simulink model "fft_wideband_real_test"  (Simulink 7.4)
settings: Solver=VariableStepDiscrete  StartTime=0.0  StopTime=150  RelTol=1e-3
libraries: xbsIndex_r4 x739, casper_library_misc x48, casper_library_delays x8, casper_library_ffts_twiddle x1, simulink x1
(part 1 of 7)
settings Model: Creator=User  LastModifiedBy=wjm
settings OptimizationCC: InitFltsAndDblsToZero=on

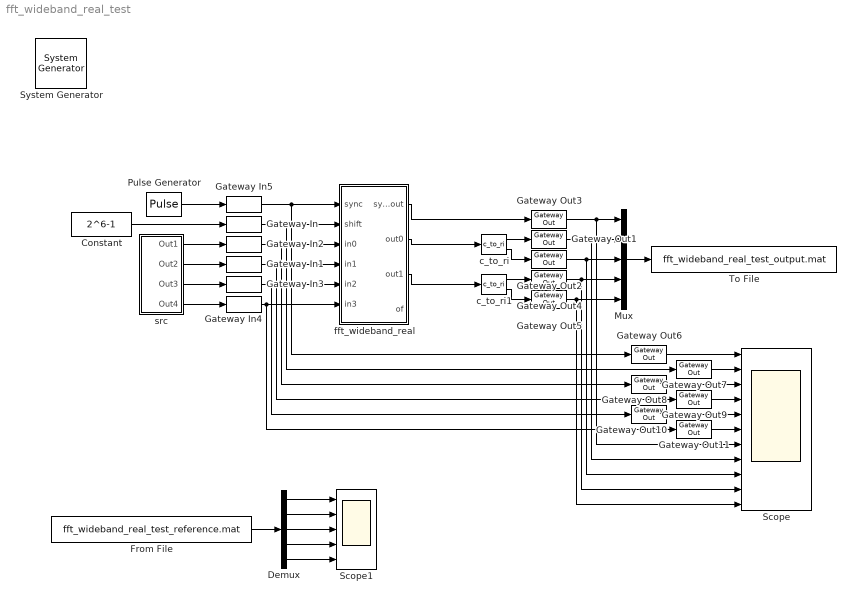
== system fft_wideband_real_test ==
  " System Generator" : xbsIndex_r4/ System Generator  Tag=genX  SystemSampleTime=-1  xilinxfamily=virtex5  part=xc5vsx95t  speed=-1  package=ff1136  synthesis_tool=XST  clock_wrapper=Clock Enables  directory=./netlist  testbench=off  simulink_period=1  sysclk_period=100  dcm_input_clock_period=100  incr_netlist=off  trim_vbits=Everywhere in SubSystem  dbl_ovrd=According to Block Masks  core_generation=According to Block Masks  run_coregen=off  deprecated_control=off  eval_field=0  block_type=sysgen
      settings: block_version=10.1.1
  Constant : Constant  Value=2^6-1  OutDataType=sfix(16)  OutScaling=2^0
  Demux : Demux  Outputs=5
  From File : FromFile  FileName=fft_wideband_real_test_reference.mat  SampleTime=1
  Gateway In : xbsIndex_r4/Gateway In  arith_type=Unsigned  n_bits=6  bin_pt=0  quantization=Truncate  overflow=Wrap  period=1  dbl_ovrd=off  timing_constraint=None  locs_specified=off  LOCs={}  hdl_port=on  block_type=gatewayin
      settings: infoedit="Gateway in block.  Converts inputs of type Simulink integer, double and fixed point to  Xilinx fixed point type.<P><P>Hardware notes:  In hardware these blocks become top level input ports."  block_version=10.1.1
  Gateway In{1..4} (4 alike) : xbsIndex_r4/Gateway In  arith_type="Signed  (2's comp)"  n_bits=12  bin_pt=11  quantization=Truncate  overflow=Wrap  period=1  dbl_ovrd=off  timing_constraint=None  locs_specified=off  LOCs={}  hdl_port=on  block_type=gatewayin
      settings: infoedit="Gateway in block.  Converts inputs of type Simulink integer, double and fixed point to  Xilinx fixed point type.<P><P>Hardware notes:  In hardware these blocks become top level input ports."  block_version=10.1.1
  Gateway In5 : xbsIndex_r4/Gateway In  arith_type=Boolean  n_bits=16  bin_pt=14  quantization="Round  (unbiased: +/- Inf)"  overflow=Saturate  period=1  dbl_ovrd=off  timing_constraint=None  locs_specified=off  LOCs={}  hdl_port=on  block_type=gatewayin
      settings: infoedit="Gateway in block.  Converts inputs of type Simulink integer, double and fixed point to  Xilinx fixed point type.<P><P>Hardware notes:  In hardware these blocks become top level input ports."  block_version=10.1.1
  Gateway Out{1..11} (11 alike) : xbsIndex_r4/Gateway Out  hdl_port=on  timing_constraint=None  locs_specified=off  LOCs={}  block_type=gatewayout
      settings: infoedit="Gateway out block.  Converts Xilinx fixed point inputs into ouputs of type Simulink integer, double, or fixed point.<P><P>Hardware notes:  In hardware these blocks become top level output ports or are discarded, depending on how they are configured."  block_version=10.1.1
  Mux : Mux  Inputs=5
  Pulse Generator : DiscretePulseGenerator  Amplitude=1  Period=2^6  PulseWidth=1  PhaseDelay=13  SampleTime=1
  Scope : Scope  NumInputPorts=11
      settings: TimeRange=256  YMin=-5~-5~-5~-5~-5~-5~-5~-5~-5~-5~-5  YMax=5~5~5~5~5~5~5~5~5~5~5
  Scope1 : Scope  NumInputPorts=5
      settings: YMin=-5~-5~-5~-5~-5  YMax=5~5~5~5~5
  To File : ToFile  Filename=fft_wideband_real_test_output.mat  MatrixName=output
  c_to_ri : casper_library_misc/c_to_ri  SystemSampleTime=-1  n_bits=12  bin_pt=11
      settings: AttributesFormatString=12_11 r/i
  c_to_ri1 : casper_library_misc/c_to_ri  SystemSampleTime=-1  n_bits=12  bin_pt=11
      settings: AttributesFormatString=12_11 r/i
  fft_wideband_real : Subsystem  AncestorBlock=casper_library_ffts/fft_wideband_real  mask(fft_wideband_real){FFTSize=5, input_bit_width=12, coeff_bit_width=12, n_inputs=2, quantization=Round  (unbiased: Even Values), overflow=Saturate, add_latency=2, mult_latency=2, bram_latency=1, conv_latency=2, arch=Virtex5, opt_target=multipliers, coeffs_bit_limit=8, delays_bit_limit=8, specify_mult=on, mult_spec=getfield( getfield( get_param( gcb,'UserData' ), 'parameters'),'mult_spec'), dsp48_adders=on}
      mask prompts: FFTSize "Size of FFT: (2^?)"; input_bit_width "Input/Output Bit Width"; coeff_bit_width "Coefficient Bit Width"; n_inputs "Number of Simultaneous Inputs: (2^?)"; quantization "Quantization Behavior"; overflow "Overflow Behavior"; add_latency "Add Latency"; mult_latency "Mult Latency"; bram_latency "BRAM Latency"; conv_latency "Convert latency"; arch "Architecture"; opt_target "Use less"; coeffs_bit_limit "Number bits above which to store stage's coefficients in BRAM (2^? bits)"; delays_bit_limit "Number bits above which to store stage's delays in BRAM (2^? bits)"; specify_mult "Specify multiplier use (behavioral HDL if not specified)"; mult_spec "Multiplier specification (0=core, 1=embedded, 2=behavioural) (left=1st stage)"; dsp48_adders "DSP48 adders in butterfly"
      mask init:
      | fft_wideband_real_init(gcb,...
      |     'FFTSize', FFTSize,...
      |     'input_bit_width', input_bit_width,...
      |     'coeff_bit_width', coeff_bit_width,...
      |     'n_inputs', n_inputs,...
      |     'quantization', quantization,...
      |     'overflow', overflow,...
      |     'add_latency', add_latency,...
      |     'mult_latency', mult_latency,...
      |     'bram_latency', bram_latency,...
      |     'conv_latency', conv_latency, ...
      |     'arch', arch, ...
      |     'opt_target', opt_target, ...
      |     'coeffs_bit_limit', coeffs_bit_limit, ...
      |     'delays_bit_limit', delays_bit_limit, ...    
      |     'specify_mult', specify_mult,...
      |     'mult_spec', mult_spec, ...
      |     'dsp48_adders', dsp48_adders);
      settings: AttributesFormatString=|
      | 5 stages
      | (12,12)
      | Round  (unbiased: Even Values)
      | Saturate
      mask Help: eval('xlWeb(''http://casper.berkeley.edu/wiki/Fft_wideband_real'')')
      mask StyleString: edit,edit,edit,edit,popup(Truncate|Round  (unbiased: +/- Inf)|Round  (unbiased: Even Values)),popup(Wrap|Saturate|Error),edit,edit,edit,edit,popup(Virtex2Pro|Virtex5),popup(logic|multipliers),edit,edit,checkbox,edit,checkbox
      mask CallbackString:
      | % fft_size = eval(get_param(gcb, 'FFTSize'));
      | % old_vec = eval(get_param(gcb, 'mult_spec'));
      | 
      | % vec = 2.*ones(1,fft_size);
      | % old_size = length(old_vec);
      | 
      | % if(old_size <= fft_size),
      | %    size = old_size;
      | % else,
      | %     size = fft_size;
      | % end
      | 
      | % for n = 1:size, vec(n) = old_vec(n); end
      | % set_param(gcb, 'mult_spec', mat2str(vec));||||||||||fft_callback_arch(gcb);||||specify_mult = get_param(gcb,'specify_mult');
      | visibs = get_param(gcb, 'MaskVisibilities');
      | enables = get_param(gcb, 'MaskEnables');
      | enables{16} = 'on';
      | if( strcmp(specify_mult,'off')), visibs{16} = 'off';
      | else, visibs{16} = 'on';
      | end
      | set_param(gcb, 'MaskEnables', enables);
      | set_param(gcb, 'MaskVisibilities', visibs);
      | |% vec = eval( get_param(gcb, 'mult_spec'));
      | % vec_size = length(vec);
      | % fft_size = eval( get_param(gcb, 'FFTSize'));
      | % new_vec = 2.*ones(1, fft_size);
      | 
      | % if(vec_size <= fft_size), size = vec_size;
      | % else size = fft_size;
      | % end
      | 
      | % for n=1:size
      | %     new_vec(n) = vec(n);
      | % end
      | % set_param(gcb, 'mult_spec', mat2str(new_vec));|fft_callback_dsp48_adders(gcb);
  src : Subsystem
  wires:
  Pulse Generator/1 -> Gateway In5/1
  Constant/1 -> Gateway In/1
  src/1(Out1) -> Gateway In2/1
  src/2(Out2) -> Gateway In1/1
  src/3(Out3) -> Gateway In3/1
  src/4(Out4) -> Gateway In4/1
  Gateway In2/1 -> Gateway Out8/1, fft_wideband_real/3(in0)
  Gateway In1/1 -> Gateway Out9/1, fft_wideband_real/4(in1)
  Gateway In3/1 -> Gateway Out10/1, fft_wideband_real/5(in2)
  Gateway In4/1 -> Gateway Out11/1, fft_wideband_real/6(in3)
  Gateway In/1 -> Gateway Out7/1, fft_wideband_real/2(shift)
  Gateway In5/1 -> Gateway Out6/1, fft_wideband_real/1(sync)
  fft_wideband_real/1(sync_out) -> Gateway Out3/1
  fft_wideband_real/2(out0) -> c_to_ri/1
  fft_wideband_real/3(out1) -> c_to_ri1/1
  c_to_ri/1 -> Gateway Out1/1
  c_to_ri/2 -> Gateway Out2/1
  c_to_ri1/1 -> Gateway Out4/1
  c_to_ri1/2 -> Gateway Out5/1
  Gateway Out3/1 -> Mux/1, Scope/7
  Gateway Out1/1 -> Mux/2, Scope/8
  Gateway Out2/1 -> Mux/3, Scope/9
  Gateway Out4/1 -> Mux/4, Scope/10
  Gateway Out5/1 -> Mux/5, Scope/11
  Mux/1 -> To File/1
  Gateway Out6/1 -> Scope/1
  Gateway Out7/1 -> Scope/2
  Gateway Out8/1 -> Scope/3
  Gateway Out9/1 -> Scope/4
  Gateway Out10/1 -> Scope/5
  Gateway Out11/1 -> Scope/6
  From File/1 -> Demux/1
  Demux/1 -> Scope1/1
  Demux/2 -> Scope1/2
  Demux/3 -> Scope1/3
  Demux/4 -> Scope1/4
  Demux/5 -> Scope1/5

== system fft_wideband_real_test/fft_wideband_real ==
  sync : Inport
  shift : Inport  Port=2
  in0 : Inport  Port=3
  in1 : Inport  Port=4
  in2 : Inport  Port=5
  in3 : Inport  Port=6
  fft_biplex_real_4x0 : Subsystem  AncestorBlock=casper_library_ffts/fft_biplex_real_4x  mask(fft_biplex_real_4x){FFTSize=3, input_bit_width=12, coeff_bit_width=12, quantization=Round  (unbiased: Even Values), overflow=Saturate, add_latency=2, mult_latency=2, bram_latency=1, conv_latency=2, arch=Virtex5, opt_target=multipliers, coeffs_bit_limit=8, delays_bit_limit=8, specify_mult=on, mult_spec=[0                                      1                                      2], dsp48_adders=on}
      mask prompts: FFTSize "Size of FFT: (2^? pnts)"; input_bit_width "Input/Output Bit Width"; coeff_bit_width "Coefficient Bit Width"; quantization "Quantization Behavior"; overflow "Overflow Behavior"; add_latency "Add Latency"; mult_latency "Mult Latency"; bram_latency "BRAM Latency"; conv_latency "Convert latency"; arch "Architecture"; opt_target "Use less"; coeffs_bit_limit "Number bits above which to store stage's coefficients in BRAM (2^? bits)"; delays_bit_limit "Number bits above which to implement stage's delays in BRAM (2^? bits)"; specify_mult "Specify multiplier use (behavioral HDL if not specified)"; mult_spec "Multiplier specification (0=core, 1=embedded, 2=behavioural) (left=1st stage)"; dsp48_adders "DSP48 adders in butterfly"
      mask init:
      | fft_biplex_real_4x_init(gcb, ...
      |     'FFTSize', FFTSize, ...
      |     'input_bit_width', input_bit_width, ...
      |     'coeff_bit_width', coeff_bit_width, ...
      |     'quantization', quantization, ...
      |     'overflow', overflow, ...
      |     'add_latency', add_latency, ...
      |     'mult_latency', mult_latency, ...
      |     'bram_latency', bram_latency, ...
      |     'conv_latency', conv_latency, ...
      |     'arch', arch, ...
      |     'opt_target', opt_target, ...
      |     'coeffs_bit_limit', coeffs_bit_limit, ...
      |     'delays_bit_limit', delays_bit_limit, ...    
      |     'specify_mult', specify_mult, ...
      |     'mult_spec', mult_spec, ...
      |     'dsp48_adders', dsp48_adders);
      settings: AttributesFormatString=|
      | Virtex5
      | 3 stages
      | [12,12]
      | Round  (unbiased: Even Values)
      | Saturate
      mask Help: eval('xlWeb(''http://casper.berkeley.edu/wiki/Fft_biplex_real_4x'')')
      mask StyleString: edit,edit,edit,popup(Truncate|Round  (unbiased: +/- Inf)|Round  (unbiased: Even Values)),popup(Wrap|Saturate|Error),edit,edit,edit,edit,popup(Virtex2Pro|Virtex5),popup(logic|multipliers),edit,edit,checkbox,edit,checkbox
      mask CallbackString:
      | % fft_size = eval(get_param(gcb, 'FFTSize'));
      | % old_vec = eval(get_param(gcb, 'mult_spec'));
      | 
      | % vec = 2.*ones(1,fft_size);
      | % old_size = length(old_vec);
      | 
      | % if(old_size <= fft_size),
      | %     size = old_size;
      | % else,
      | %     size = fft_size;
      | % end
      | 
      | % for n = 1:size, vec(n) = old_vec(n); end
      | % set_param(gcb, 'mult_spec', mat2str(vec));|||||||||fft_callback_arch(gcb);||||specify_mult = get_param(gcb,'specify_mult');
      | visibs = get_param(gcb, 'MaskVisibilities');
      | enables = get_param(gcb, 'MaskEnables');
      | enables{15} = 'on';
      | if( strcmp(specify_mult,'off')), visibs{15} = 'off';
      | else, visibs{15} = 'on';
      | end
      | set_param(gcb, 'MaskVisibilities', visibs);
      | set_param(gcb, 'MaskEnables', enables);
      | |% vec = eval( get_param(gcb, 'mult_spec'));
      | % vec_size = length(vec);
      | % fft_size = eval( get_param(gcb, 'FFTSize'));
      | % new_vec = 2.*ones(1, fft_size);
      | 
      | % if(vec_size <= fft_size), size = vec_size;
      | % else size = fft_size;
      | % end
      | 
      | % for n=1:size
      | %    new_vec(n) = vec(n);
      | % end
      | % set_param(gcb, 'mult_spec', mat2str(new_vec));|fft_callback_dsp48_adders(gcb);
  fft_direct : Subsystem  AncestorBlock=casper_library_ffts/fft_direct  mask(fft_direct){FFTSize=2, input_bit_width=12, coeff_bit_width=12, add_latency=2, mult_latency=2, bram_latency=1, conv_latency=2, quantization=Round  (unbiased: Even Values), overflow=Saturate, map_tail=on, LargerFFTSize=5, StartStage=4, arch=Virtex5, opt_target=multipliers, coeffs_bit_limit=8, specify_mult=on, mult_spec=[0                                      1], dsp48_adders=on}
      mask prompts: FFTSize "Size of FFT: (2^?)"; input_bit_width "Input/Output Bit Width"; coeff_bit_width "Coefficient Bit Width"; add_latency "Add Latency"; mult_latency "Mult Latency"; bram_latency "BRAM Latency"; conv_latency "Convert latency"; quantization "Quantization Behavior"; overflow "Overflow Behavior"; map_tail "Map Tail of Larger FFT"; LargerFFTSize "Size of Larger FFT (2^?):"; StartStage "Start Stage of Map Tail:"; arch "Architecture"; opt_target "Use less"; coeffs_bit_limit "Number bits above which to store stage's coefficients in BRAM (2^? bits)"; specify_mult "Specify multiplier use (behavioural HDL if not specified)"; mult_spec "Multiplier specification (0=core, 1=behavioural HDL, 2=embedded) (left=1st stage)"; dsp48_adders "DSP48 adders in butterfly"
      mask help:
      | Implements an N-point FFT with the classic
      | butterfly structure with N inputs and N outputs
      mask init:
      | fft_direct_init(gcb,...
      |     'FFTSize', FFTSize, ...
      |     'input_bit_width', input_bit_width, ...
      |     'coeff_bit_width', coeff_bit_width, ...
      |     'add_latency', add_latency, ...
      |     'mult_latency', mult_latency, ...
      |     'bram_latency', bram_latency, ...
      |     'conv_latency', conv_latency, ...
      |     'quantization', quantization, ...
      |     'overflow', overflow, ...
      |     'map_tail', map_tail, ...
      |     'LargerFFTSize', LargerFFTSize, ...
      |     'StartStage', StartStage, ...
      |     'arch', arch, ...
      |     'opt_target', opt_target, ...
      |     'coeffs_bit_limit', coeffs_bit_limit, ...
      |     'specify_mult', specify_mult, ...
      |     'mult_spec', mult_spec, ...
      |     'dsp48_adders', dsp48_adders);
      settings: AttributesFormatString=|
      | Virtex5
      | stages [4  5] of 5
      | [12,12]
      | Round  (unbiased: Even Values)
      | Saturate
      mask StyleString: edit,edit,edit,edit,edit,edit,edit,popup(Truncate|Round  (unbiased: +/- Inf)|Round  (unbiased: Even Values)),popup(Wrap|Saturate|Error),checkbox,edit,edit,popup(Virtex2Pro|Virtex5),popup(logic|multipliers),edit,checkbox,edit,checkbox
      mask CallbackString:
      | % fft_size = eval(get_param(gcb, 'FFTSize'));
      | % old_vec = eval(get_param(gcb, 'mult_spec'));
      | 
      | % vec = 2.*ones(1,fft_size);
      | % old_size = length(old_vec);
      | 
      | % if(old_size <= fft_size),
      | %     size = old_size;
      | % else,
      | %     size = fft_size;
      | % end
      | 
      | % for n = 1:size, vec(n) = old_vec(n); end
      | % set_param(gcb, 'mult_spec', mat2str(vec));|||||||||map_tail = get_param(gcb,'map_tail');
      | visibs = get_param(gcb, 'MaskVisibilities');
      | if( strcmp(map_tail,'off')),
      |     visibs{11} = 'off';
      |     visibs{12} = 'off';
      | else,
      |     visibs{11} = 'on';
      |     visibs{12} = 'on';
      | end
      | set_param(gcb, 'MaskVisibilities', visibs);
      | |||fft_callback_arch(gcb);|||specify_mult = get_param(gcb,'specify_mult');
      | visibs = get_param(gcb, 'MaskVisibilities');
      | if( strcmp(specify_mult,'off')), visibs{17} = 'off';
      | else, visibs{17} = 'on';
      | end
      | set_param(gcb, 'MaskVisibilities', visibs);
      | |% vec = eval( get_param(gcb, 'mult_spec'));
      | % vec_size = length(vec);
      | % fft_size = eval( get_param(gcb, 'FFTSize'));
      | % new_vec = 2.*ones(1, fft_size);
      | 
      | % if(vec_size <= fft_size), size = vec_size;
      | % else size = fft_size;
      | % end
      | 
      | % for n=1:size
      | %     new_vec(n) = vec(n);
      | % end
      | % set_param(gcb, 'mult_spec', mat2str(new_vec));|fft_callback_dsp48_adders(gcb);
  fft_unscrambler : Subsystem  AncestorBlock=casper_library_ffts/fft_unscrambler  mask(fft_unscrambler){FFTSize=4, n_inputs=1, bram_latency=1}
      mask prompts: FFTSize "Size of FFT: (2^?)"; n_inputs "Number of Simultaneous Inputs: (2^?)"; bram_latency "BRAM Latency"
      mask init:
      | fft_unscrambler_init(gcb,...
      |     'FFTSize',FFTSize,... 
      |     'n_inputs', n_inputs,...
      |     'bram_latency', bram_latency);
      settings: AttributesFormatString=FFTSize=4, n_inputs=1
  of_or : xbsIndex_r4/Logical  logical_function=OR  inputs=2  en=off  latency=1  precision=Full  arith_type=Unsigned  n_bits=16  bin_pt=0  align_bp=on  dbl_ovrd=off  block_type=logical
      settings: block_version=11.4
  slice : xbsIndex_r4/Slice  nbits=2  boolean_output=off  mode=Lower Bit Location + Width  bit1=0  base1=MSB of Input  bit0=3  base0=LSB of Input  dbl_ovrd=off  block_type=slice
  sync_out : Outport
  out0 : Outport  Port=2
  out1 : Outport  Port=3
  of : Outport  Port=4
  wires:
  in0/1 -> fft_biplex_real_4x0/1(pol1)
  in1/1 -> fft_biplex_real_4x0/2(pol2)
  in2/1 -> fft_biplex_real_4x0/3(pol3)
  in3/1 -> fft_biplex_real_4x0/4(pol4)
  shift/1 -> fft_biplex_real_4x0/6(shift), slice/1
  sync/1 -> fft_biplex_real_4x0/5(sync)
  fft_biplex_real_4x0/5(of) -> of_or/2
  slice/1 -> fft_direct/2(shift)
  fft_biplex_real_4x0/6(sync_out) -> fft_direct/1(sync)
  fft_biplex_real_4x0/1(pol1_out) -> fft_direct/3(in0)
  fft_biplex_real_4x0/2(pol2_out) -> fft_direct/4(in1)
  fft_biplex_real_4x0/3(pol3_out) -> fft_direct/5(in2)
  fft_biplex_real_4x0/4(pol4_out) -> fft_direct/6(in3)
  fft_direct/6(of) -> of_or/1
  of_or/1 -> of/1
  fft_direct/1(sync_out) -> fft_unscrambler/1(sync)
  fft_unscrambler/1(sync_out) -> sync_out/1
  fft_direct/2(out0) -> fft_unscrambler/2(In1)
  fft_unscrambler/2(Out1) -> out0/1
  fft_direct/3(out1) -> fft_unscrambler/3(In2)
  fft_unscrambler/3(Out2) -> out1/1

== system fft_wideband_real_test/src ==
  Band-Limited White Noise : simulink/Sources/Band-Limited White Noise  SystemSampleTime=-1  Cov=[0.001]  Ts=1  seed=[23341]
  Constant : Constant  Value=0  OutDataType=sfix(16)  OutScaling=2^0
  Pulse Generator1 : DiscretePulseGenerator  Amplitude=0.75  Period=2^5  PulseWidth=1  PhaseDelay=14  SampleTime=1
  Pulse Generator2 : DiscretePulseGenerator  Amplitude=0.5  Period=2^6  PulseWidth=1  PhaseDelay=15  SampleTime=1
  Sine Wave : Sin  SineType=Sample based  Amplitude=0.125  Bias=0  Frequency=1  Phase=0  Samples=8  SampleTime=1  Offset=0
  Out1 : Outport
  Out2 : Outport  Port=2
  Out3 : Outport  Port=3
  Out4 : Outport  Port=4
  wires:
  Pulse Generator2/1 -> Out4/1, Out3/1
  Pulse Generator1/1 -> Out1/1, Out2/1

== system fft_wideband_real_test/fft_wideband_real/fft_biplex_real_4x0 ==
  pol1 : Inport  OutDataType=sfix(16)  OutScaling=2^0
  pol2 : Inport  Port=2  OutDataType=sfix(16)  OutScaling=2^0
  pol3 : Inport  Port=3  OutDataType=sfix(16)  OutScaling=2^0
  pol4 : Inport  Port=4  OutDataType=sfix(16)  OutScaling=2^0
  sync : Inport  Port=5  OutDataType=sfix(16)  OutScaling=2^0
  shift : Inport  Port=6  OutDataType=sfix(16)  OutScaling=2^0
  bi_real_unscr_4x : Subsystem  mask{FFTSize=3, bram_latency=1}
      mask prompts: FFTSize "Size of FFT (2^?):"; bram_latency "BRAM Latency"
      mask init:
      | blk = gcb;
      | if same_state(blk, 'FFTSize', FFTSize, 'bram_latency', bram_latency), return, end
      | set_param([blk,'/reorder'],'map', mat2str(bit_reverse(0:2^(FFTSize-1)-1, FFTSize-1)));
      | set_param([blk,'/reorder'],'bram_latency', num2str(bram_latency));
      | set_param([blk,'/reorder1'],'map', mat2str(bit_reverse(2^(FFTSize-1)-1:-1:0, FFTSize-1)));
      | set_param([blk,'/reorder1'],'bram_latency', num2str(bram_latency));
      | set_param([blk,'/reorder2'],'map', mat2str(2^(FFTSize-1)-1:-1:0));
      | set_param([blk,'/reorder2'],'bram_latency', num2str(bram_latency));
      | save_state(blk, 'FFTSize', FFTSize, 'bram_latency', bram_latency);
  biplex_core : Subsystem  AncestorBlock=casper_library_ffts/biplex_core  mask(biplex_core){FFTSize=3, input_bit_width=12, coeff_bit_width=12, quantization=Round  (unbiased: Even Values), overflow=Saturate, add_latency=2, mult_latency=2, bram_latency=1, conv_latency=2, arch=Virtex5, opt_target=multipliers, coeffs_bit_limit=8, delays_bit_limit=8, specify_mult=on, mult_spec=[0                                      1                                      2], dsp48_adders=on}
      mask prompts: FFTSize "Size of FFT: (2^? pnts)"; input_bit_width "Input/Output Bit Width"; coeff_bit_width "Coefficient Bit Width"; quantization "Quantization Behavior"; overflow "Overflow Behavior"; add_latency "Add Latency"; mult_latency "Mult Latency"; bram_latency "BRAM Latency"; conv_latency "Convert latency"; arch "Architecture"; opt_target "Use less"; coeffs_bit_limit "Number bits above which to store stage's coefficients in BRAM (2^? bits)"; delays_bit_limit "Number bits above which to implent stage's delays in BRAM (2^? bits)"; specify_mult "Specify multiplier use (behavioural HDL if not specified)"; mult_spec "Multiplier specification (0=core, 1=embedded, 2=behavioural) (left=1st stage)"; dsp48_adders "Use DSP48s for adders"
      mask init:
      | biplex_core_init(gcb,...
      |     'FFTSize', FFTSize,...
      |     'input_bit_width', input_bit_width,...
      |     'coeff_bit_width', coeff_bit_width,...
      |     'quantization', quantization,...
      |     'overflow', overflow,...
      |     'add_latency', add_latency,...
      |     'mult_latency', mult_latency,...
      |     'bram_latency', bram_latency,...
      |     'conv_latency', conv_latency, ...
      |     'arch', arch, ...
      |     'opt_target', opt_target, ...
      |     'coeffs_bit_limit', coeffs_bit_limit, ...
      |     'delays_bit_limit', delays_bit_limit, ...
      |     'specify_mult', specify_mult, ...
      |     'mult_spec', mult_spec, ...
      |     'dsp48_adders', dsp48_adders );
      settings: AttributesFormatString=|
      | 3 stages
      | reduce multipliers
      | Virtex5
      mask StyleString: edit,edit,edit,popup(Truncate|Round  (unbiased: +/- Inf)|Round  (unbiased: Even Values)),popup(Wrap|Saturate|Error),edit,edit,edit,edit,popup(Virtex2Pro|Virtex5),popup(logic|multipliers),edit,edit,checkbox,edit,checkbox
      mask CallbackString:
      | % fft_size = eval(get_param(gcb, 'FFTSize'));
      | % old_vec = eval(get_param(gcb, 'mult_spec'));
      | 
      | % vec = 2.*ones(1,fft_size);
      | % old_size = length(old_vec);
      | 
      | % if(old_size <= fft_size),
      | %    size = old_size;
      | % else,
      | %     size = fft_size;
      | % end
      | 
      | % for n = 1:size, vec(n) = old_vec(n); end
      | % set_param(gcb, 'mult_spec', mat2str(vec));|||||||||fft_callback_arch(gcb);||||specify_mult = get_param(gcb,'specify_mult');
      | visibs = get_param(gcb,'MaskVisibilities');
      | if( strcmp(specify_mult,'off')), visibs{15} = 'off';
      | else, visibs{15} = 'on';
      | end
      | set_param(gcb, 'MaskVisibilities', visibs);
      | enables = get_param(gcb,'MaskVisibilities');
      | enables{15} = 'on';
      | set_param(gcb, 'MaskEnables', enables);
      | |% vec = eval( get_param(gcb, 'mult_spec'));
      | % vec_size = length(vec);
      | % fft_size = eval( get_param(gcb, 'FFTSize'));
      | % new_vec = 2.*ones(1, fft_size);
      | 
      | % if(vec_size <= fft_size), size = vec_size;
      | % else size = fft_size;
      | % end
      | 
      | % for n=1:size
      | %     new_vec(n) = vec(n);
      | % end
      | % set_param(gcb, 'mult_spec', mat2str(new_vec));|fft_callback_dsp48_adders(gcb);
  ri_to_c : Subsystem
  ri_to_c1 : Subsystem
  pol1_out : Outport  OutDataType=sfix(16)  OutScaling=2^0
  pol2_out : Outport  Port=2  OutDataType=sfix(16)  OutScaling=2^0
  pol3_out : Outport  Port=3  OutDataType=sfix(16)  OutScaling=2^0
  pol4_out : Outport  Port=4  OutDataType=sfix(16)  OutScaling=2^0
  of : Outport  Port=5  OutDataType=sfix(16)  OutScaling=2^0
  sync_out : Outport  Port=6  OutDataType=sfix(16)  OutScaling=2^0
  wires:
  bi_real_unscr_4x/5(sync_out) -> sync_out/1
  bi_real_unscr_4x/4(pol4_out) -> pol4_out/1
  bi_real_unscr_4x/3(pol3_out) -> pol3_out/1
  bi_real_unscr_4x/2(pol2_out) -> pol2_out/1
  bi_real_unscr_4x/1(pol1_out) -> pol1_out/1
  shift/1 -> biplex_core/4(shift)
  sync/1 -> biplex_core/3(sync)
  pol4/1 -> ri_to_c1/2(im)
  ri_to_c1/1(c) -> biplex_core/2(pol2)
  pol3/1 -> ri_to_c1/1(re)
  pol2/1 -> ri_to_c/2(im)
  ri_to_c/1(c) -> biplex_core/1(pol1)
  pol1/1 -> ri_to_c/1(re)
  biplex_core/3(of) -> of/1
  biplex_core/1(out1) -> bi_real_unscr_4x/1(even)
  biplex_core/2(out2) -> bi_real_unscr_4x/2(odd)
  biplex_core/4(sync_out) -> bi_real_unscr_4x/3(sync)

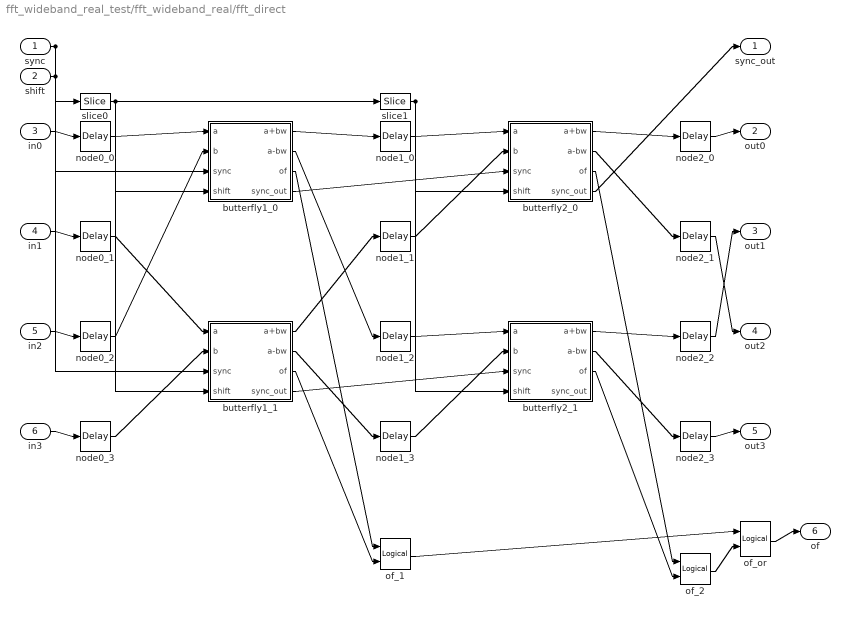
== system fft_wideband_real_test/fft_wideband_real/fft_direct ==
  sync : Inport
  shift : Inport  Port=2
  in0 : Inport  Port=3
  in1 : Inport  Port=4
  in2 : Inport  Port=5
  in3 : Inport  Port=6
  butterfly1_0 : Subsystem  AncestorBlock=casper_library_ffts/butterfly_direct  mask(butterfly_direct){biplex=off, FFTSize=5, Coeffs=getfield( getfield( get_param( gcb,'UserData' ), 'parameters'),'Coeffs'), StepPeriod=0, coeffs_bram=off, coeff_bit_width=12, input_bit_width=12, bram_latency=1, add_latency=2, mult_latency=2, conv_latency=2, quantization=Round  (unbiased: Even Values), overflow=Saturate, arch=Virtex5, opt_target=multipliers, use_hdl=off, use_embedded=off, dsp48_adders=on}
      mask prompts: biplex "Used in biplex FFT"; FFTSize "Size of FFT: (2^?)"; Coeffs "Coefficients: (0 to 2^(FFTSize-1)-1)"; StepPeriod "Coefficient Step Period: (2^?)"; coeffs_bram "Implement coefficients in BRAM"; coeff_bit_width "Coefficient Bit Width"; input_bit_width "Input/Output Bit Width:"; bram_latency "BRAM Latency"; add_latency "Add Latency"; mult_latency "Mult Latency"; conv_latency "Convert latency"; quantization "Quantization Behavior"; overflow "Overflow Behavior"; arch "Architecture"; opt_target "Use less"; use_hdl "Use behavioural HDL for multipliers"; use_embedded "Use embedded multipliers"; dsp48_adders "Use DSP48s for adders"
      mask init:
      | butterfly_direct_init(gcb,...
      |     'biplex', biplex,...
      |     'FFTSize', FFTSize,...
      |     'Coeffs', Coeffs,...
      |     'coeff_bit_width', coeff_bit_width,...
      |     'StepPeriod', StepPeriod,...
      |     'input_bit_width', input_bit_width,...
      |     'add_latency', add_latency,...
      |     'mult_latency', mult_latency,...
      |     'bram_latency', bram_latency,...
      |     'conv_latency', conv_latency, ...
      |     'coeffs_bram', coeffs_bram,...    
      |     'quantization', quantization,...
      |     'overflow', overflow,...
      |     'arch', arch,...
      |     'opt_target', opt_target,...
      |     'use_hdl', use_hdl,...
      |     'use_embedded', use_embedded,...
      |     'dsp48_adders', dsp48_adders);
      settings: AttributesFormatString=|
      | twiddle_general_3mult
      | coeffs in slices
      mask StyleString: checkbox,edit,edit,edit,checkbox,edit,edit,edit,edit,edit,edit,popup(Truncate|Round  (unbiased: +/- Inf)|Round  (unbiased: Even Values)),popup(Wrap|Saturate|Error),popup(Virtex2Pro|Virtex5),popup(logic|multipliers),checkbox,checkbox,checkbox
      mask CallbackString:
      | ||%coeffs = eval(get_param(gcb,'Coeffs'));
      | %visibs = get_param(gcb,'MaskVisibilities');
      | %if length(coeffs) == 1,
      | %    visibs{4} = 'off'; visibs{5} = 'off';
      | %    visibs{6} = 'off';
      | %else
      | %    visibs{4} = 'on';
      | %    visibs{5} = 'on'; visibs{6} = 'on';
      | %end
      | %set_param(gcb, 'MaskVisibilities', visibs);|%coeffs = eval(get_param(gcb,'Coeffs'));
      | %visibs = get_param(gcb,'MaskVisibilities');
      | %if length(coeffs) == 1,
      | %    visibs{4} = 'off'; visibs{5} = 'off';
      | %    visibs{6} = 'off';
      | %else
      | %%    visibs{4} = 'on';
      | %    visibs{5} = 'on'; visibs{6} = 'on';
      | %end
      | %set_param(gcb, 'MaskVisibilities', visibs);|%coeffs = eval(get_param(gcb,'Coeffs'));
      | %visibs = get_param(gcb,'MaskVisibilities');
      | %if length(coeffs) == 1,
      | %    visibs{5} = 'off'; visibs{6} = 'off';
      | %    visibs{7} = 'off';
      | %else
      | %    visibs{5} = 'on';
      | %    visibs{6} = 'on'; visibs{7} = 'on';
      | %end
      | %set_param(gcb, 'MaskVisibilities', visibs);|||||||||fft_callback_arch(gcb);||use_hdl = get_param(gcb,'use_hdl');
      | visibs = get_param(gcb, 'MaskVisibilities');
      | if( strcmp(use_hdl,'on')),
      |     set_param(gcb, 'use_embedded','off');
      |     visibs{17} = 'off';
      | else,
      |     visibs{17} = 'on';
      | end
      |     set_param(gcb, 'MaskVisibilities',visibs);||fft_callback_dsp48_adders(gcb);
  butterfly1_1 : Subsystem  AncestorBlock=casper_library_ffts/butterfly_direct  mask(butterfly_direct){biplex=off, FFTSize=5, Coeffs=getfield( getfield( get_param( gcb,'UserData' ), 'parameters'),'Coeffs'), StepPeriod=0, coeffs_bram=off, coeff_bit_width=12, input_bit_width=12, bram_latency=1, add_latency=2, mult_latency=2, conv_latency=2, quantization=Round  (unbiased: Even Values), overflow=Saturate, arch=Virtex5, opt_target=multipliers, use_hdl=off, use_embedded=off, dsp48_adders=on}
      mask prompts: biplex "Used in biplex FFT"; FFTSize "Size of FFT: (2^?)"; Coeffs "Coefficients: (0 to 2^(FFTSize-1)-1)"; StepPeriod "Coefficient Step Period: (2^?)"; coeffs_bram "Implement coefficients in BRAM"; coeff_bit_width "Coefficient Bit Width"; input_bit_width "Input/Output Bit Width:"; bram_latency "BRAM Latency"; add_latency "Add Latency"; mult_latency "Mult Latency"; conv_latency "Convert latency"; quantization "Quantization Behavior"; overflow "Overflow Behavior"; arch "Architecture"; opt_target "Use less"; use_hdl "Use behavioural HDL for multipliers"; use_embedded "Use embedded multipliers"; dsp48_adders "Use DSP48s for adders"
      mask init: same as fft_wideband_real_test/fft_wideband_real/fft_direct/butterfly1_0
      settings: AttributesFormatString=|
      | twiddle_general_3mult
      | coeffs in slices
      mask StyleString: checkbox,edit,edit,edit,checkbox,edit,edit,edit,edit,edit,edit,popup(Truncate|Round  (unbiased: +/- Inf)|Round  (unbiased: Even Values)),popup(Wrap|Saturate|Error),popup(Virtex2Pro|Virtex5),popup(logic|multipliers),checkbox,checkbox,checkbox
      mask CallbackString:
      | ||%coeffs = eval(get_param(gcb,'Coeffs'));
      | %visibs = get_param(gcb,'MaskVisibilities');
      | %if length(coeffs) == 1,
      | %    visibs{4} = 'off'; visibs{5} = 'off';
      | %    visibs{6} = 'off';
      | %else
      | %    visibs{4} = 'on';
      | %    visibs{5} = 'on'; visibs{6} = 'on';
      | %end
      | %set_param(gcb, 'MaskVisibilities', visibs);|%coeffs = eval(get_param(gcb,'Coeffs'));
      | %visibs = get_param(gcb,'MaskVisibilities');
      | %if length(coeffs) == 1,
      | %    visibs{4} = 'off'; visibs{5} = 'off';
      | %    visibs{6} = 'off';
      | %else
      | %%    visibs{4} = 'on';
      | %    visibs{5} = 'on'; visibs{6} = 'on';
      | %end
      | %set_param(gcb, 'MaskVisibilities', visibs);|%coeffs = eval(get_param(gcb,'Coeffs'));
      | %visibs = get_param(gcb,'MaskVisibilities');
      | %if length(coeffs) == 1,
      | %    visibs{5} = 'off'; visibs{6} = 'off';
      | %    visibs{7} = 'off';
      | %else
      | %    visibs{5} = 'on';
      | %    visibs{6} = 'on'; visibs{7} = 'on';
      | %end
      | %set_param(gcb, 'MaskVisibilities', visibs);|||||||||fft_callback_arch(gcb);||use_hdl = get_param(gcb,'use_hdl');
      | visibs = get_param(gcb, 'MaskVisibilities');
      | if( strcmp(use_hdl,'on')),
      |     set_param(gcb, 'use_embedded','off');
      |     visibs{17} = 'off';
      | else,
      |     visibs{17} = 'on';
      | end
      |     set_param(gcb, 'MaskVisibilities',visibs);||fft_callback_dsp48_adders(gcb);
  butterfly2_0 : Subsystem  AncestorBlock=casper_library_ffts/butterfly_direct  mask(butterfly_direct){biplex=off, FFTSize=5, Coeffs=getfield( getfield( get_param( gcb,'UserData' ), 'parameters'),'Coeffs'), StepPeriod=0, coeffs_bram=off, coeff_bit_width=12, input_bit_width=12, bram_latency=1, add_latency=2, mult_latency=2, conv_latency=2, quantization=Round  (unbiased: Even Values), overflow=Saturate, arch=Virtex5, opt_target=multipliers, use_hdl=off, use_embedded=on, dsp48_adders=on}
      mask prompts: biplex "Used in biplex FFT"; FFTSize "Size of FFT: (2^?)"; Coeffs "Coefficients: (0 to 2^(FFTSize-1)-1)"; StepPeriod "Coefficient Step Period: (2^?)"; coeffs_bram "Implement coefficients in BRAM"; coeff_bit_width "Coefficient Bit Width"; input_bit_width "Input/Output Bit Width:"; bram_latency "BRAM Latency"; add_latency "Add Latency"; mult_latency "Mult Latency"; conv_latency "Convert latency"; quantization "Quantization Behavior"; overflow "Overflow Behavior"; arch "Architecture"; opt_target "Use less"; use_hdl "Use behavioural HDL for multipliers"; use_embedded "Use embedded multipliers"; dsp48_adders "Use DSP48s for adders"
      mask init: same as fft_wideband_real_test/fft_wideband_real/fft_direct/butterfly1_0
      settings: AttributesFormatString=|
      | twiddle_general_3mult
      | coeffs in slices
      mask StyleString: checkbox,edit,edit,edit,checkbox,edit,edit,edit,edit,edit,edit,popup(Truncate|Round  (unbiased: +/- Inf)|Round  (unbiased: Even Values)),popup(Wrap|Saturate|Error),popup(Virtex2Pro|Virtex5),popup(logic|multipliers),checkbox,checkbox,checkbox
      mask CallbackString:
      | ||%coeffs = eval(get_param(gcb,'Coeffs'));
      | %visibs = get_param(gcb,'MaskVisibilities');
      | %if length(coeffs) == 1,
      | %    visibs{4} = 'off'; visibs{5} = 'off';
      | %    visibs{6} = 'off';
      | %else
      | %    visibs{4} = 'on';
      | %    visibs{5} = 'on'; visibs{6} = 'on';
      | %end
      | %set_param(gcb, 'MaskVisibilities', visibs);|%coeffs = eval(get_param(gcb,'Coeffs'));
      | %visibs = get_param(gcb,'MaskVisibilities');
      | %if length(coeffs) == 1,
      | %    visibs{4} = 'off'; visibs{5} = 'off';
      | %    visibs{6} = 'off';
      | %else
      | %%    visibs{4} = 'on';
      | %    visibs{5} = 'on'; visibs{6} = 'on';
      | %end
      | %set_param(gcb, 'MaskVisibilities', visibs);|%coeffs = eval(get_param(gcb,'Coeffs'));
      | %visibs = get_param(gcb,'MaskVisibilities');
      | %if length(coeffs) == 1,
      | %    visibs{5} = 'off'; visibs{6} = 'off';
      | %    visibs{7} = 'off';
      | %else
      | %    visibs{5} = 'on';
      | %    visibs{6} = 'on'; visibs{7} = 'on';
      | %end
      | %set_param(gcb, 'MaskVisibilities', visibs);|||||||||fft_callback_arch(gcb);||use_hdl = get_param(gcb,'use_hdl');
      | visibs = get_param(gcb, 'MaskVisibilities');
      | if( strcmp(use_hdl,'on')),
      |     set_param(gcb, 'use_embedded','off');
      |     visibs{17} = 'off';
      | else,
      |     visibs{17} = 'on';
      | end
      |     set_param(gcb, 'MaskVisibilities',visibs);||fft_callback_dsp48_adders(gcb);
  butterfly2_1 : Subsystem  AncestorBlock=casper_library_ffts/butterfly_direct  mask(butterfly_direct){biplex=off, FFTSize=5, Coeffs=getfield( getfield( get_param( gcb,'UserData' ), 'parameters'),'Coeffs'), StepPeriod=0, coeffs_bram=off, coeff_bit_width=12, input_bit_width=12, bram_latency=1, add_latency=2, mult_latency=2, conv_latency=2, quantization=Round  (unbiased: Even Values), overflow=Saturate, arch=Virtex5, opt_target=multipliers, use_hdl=off, use_embedded=on, dsp48_adders=on}
      mask prompts: biplex "Used in biplex FFT"; FFTSize "Size of FFT: (2^?)"; Coeffs "Coefficients: (0 to 2^(FFTSize-1)-1)"; StepPeriod "Coefficient Step Period: (2^?)"; coeffs_bram "Implement coefficients in BRAM"; coeff_bit_width "Coefficient Bit Width"; input_bit_width "Input/Output Bit Width:"; bram_latency "BRAM Latency"; add_latency "Add Latency"; mult_latency "Mult Latency"; conv_latency "Convert latency"; quantization "Quantization Behavior"; overflow "Overflow Behavior"; arch "Architecture"; opt_target "Use less"; use_hdl "Use behavioural HDL for multipliers"; use_embedded "Use embedded multipliers"; dsp48_adders "Use DSP48s for adders"
      mask init: same as fft_wideband_real_test/fft_wideband_real/fft_direct/butterfly1_0
      settings: AttributesFormatString=|
      | twiddle_general_3mult
      | coeffs in slices
      mask StyleString: checkbox,edit,edit,edit,checkbox,edit,edit,edit,edit,edit,edit,popup(Truncate|Round  (unbiased: +/- Inf)|Round  (unbiased: Even Values)),popup(Wrap|Saturate|Error),popup(Virtex2Pro|Virtex5),popup(logic|multipliers),checkbox,checkbox,checkbox
      mask CallbackString:
      | ||%coeffs = eval(get_param(gcb,'Coeffs'));
      | %visibs = get_param(gcb,'MaskVisibilities');
      | %if length(coeffs) == 1,
      | %    visibs{4} = 'off'; visibs{5} = 'off';
      | %    visibs{6} = 'off';
      | %else
      | %    visibs{4} = 'on';
      | %    visibs{5} = 'on'; visibs{6} = 'on';
      | %end
      | %set_param(gcb, 'MaskVisibilities', visibs);|%coeffs = eval(get_param(gcb,'Coeffs'));
      | %visibs = get_param(gcb,'MaskVisibilities');
      | %if length(coeffs) == 1,
      | %    visibs{4} = 'off'; visibs{5} = 'off';
      | %    visibs{6} = 'off';
      | %else
      | %%    visibs{4} = 'on';
      | %    visibs{5} = 'on'; visibs{6} = 'on';
      | %end
      | %set_param(gcb, 'MaskVisibilities', visibs);|%coeffs = eval(get_param(gcb,'Coeffs'));
      | %visibs = get_param(gcb,'MaskVisibilities');
      | %if length(coeffs) == 1,
      | %    visibs{5} = 'off'; visibs{6} = 'off';
      | %    visibs{7} = 'off';
      | %else
      | %    visibs{5} = 'on';
      | %    visibs{6} = 'on'; visibs{7} = 'on';
      | %end
      | %set_param(gcb, 'MaskVisibilities', visibs);|||||||||fft_callback_arch(gcb);||use_hdl = get_param(gcb,'use_hdl');
      | visibs = get_param(gcb, 'MaskVisibilities');
      | if( strcmp(use_hdl,'on')),
      |     set_param(gcb, 'use_embedded','off');
      |     visibs{17} = 'off';
      | else,
      |     visibs{17} = 'on';
      | end
      |     set_param(gcb, 'MaskVisibilities',visibs);||fft_callback_dsp48_adders(gcb);
  node0_{0..3} (4 alike) : xbsIndex_r4/Delay  en=off  latency=0  dbl_ovrd=off  reg_retiming=off  block_type=delay
      settings: block_version=11.4
  node1_{0..3} (4 alike) : xbsIndex_r4/Delay  en=off  latency=0  dbl_ovrd=off  reg_retiming=off  block_type=delay
      settings: block_version=11.4
  node2_{0..3} (4 alike) : xbsIndex_r4/Delay  en=off  latency=0  dbl_ovrd=off  reg_retiming=off  block_type=delay
      settings: block_version=11.4
  of_1 : xbsIndex_r4/Logical  logical_function=OR  inputs=2  en=off  latency=1  precision=Full  arith_type=Unsigned  n_bits=16  bin_pt=0  align_bp=on  dbl_ovrd=off  block_type=logical
      settings: block_version=11.4
  of_2 : xbsIndex_r4/Logical  logical_function=OR  inputs=2  en=off  latency=1  precision=Full  arith_type=Unsigned  n_bits=16  bin_pt=0  align_bp=on  dbl_ovrd=off  block_type=logical
      settings: block_version=11.4
  of_or : xbsIndex_r4/Logical  logical_function=OR  inputs=2  en=off  latency=0  precision=Full  arith_type=Unsigned  n_bits=16  bin_pt=0  align_bp=on  dbl_ovrd=off  block_type=logical
      settings: block_version=11.4
  slice0 : xbsIndex_r4/Slice  nbits=1  boolean_output=on  mode=Lower Bit Location + Width  bit1=0  base1=MSB of Input  bit0=0  base0=LSB of Input  dbl_ovrd=off  block_type=slice
  slice1 : xbsIndex_r4/Slice  nbits=1  boolean_output=on  mode=Lower Bit Location + Width  bit1=0  base1=MSB of Input  bit0=1  base0=LSB of Input  dbl_ovrd=off  block_type=slice
  sync_out : Outport
  out0 : Outport  Port=2
  out1 : Outport  Port=3
  out2 : Outport  Port=4
  out3 : Outport  Port=5
  of : Outport  Port=6
  wires:
  of_or/1 -> of/1
  in0/1 -> node0_0/1
  in1/1 -> node0_1/1
  in2/1 -> node0_2/1
  in3/1 -> node0_3/1
  shift/1 -> slice0/1, slice1/1
  node2_0/1 -> out0/1
  node2_1/1 -> out2/1
  node2_2/1 -> out1/1
  node2_3/1 -> out3/1
  of_1/1 -> of_or/1
  node0_0/1 -> butterfly1_0/1(a)
  node0_2/1 -> butterfly1_0/2(b)
  butterfly1_0/1(a+bw) -> node1_0/1
  butterfly1_0/2(a-bw) -> node1_2/1
  sync/1 -> butterfly1_0/3(sync), butterfly1_1/3(sync)
  slice0/1 -> butterfly1_0/4(shift), butterfly1_1/4(shift)
  butterfly1_0/3(of) -> of_1/1
  node0_1/1 -> butterfly1_1/1(a)
  node0_3/1 -> butterfly1_1/2(b)
  butterfly1_1/1(a+bw) -> node1_1/1
  butterfly1_1/2(a-bw) -> node1_3/1
  butterfly1_1/3(of) -> of_1/2
  of_2/1 -> of_or/2
  node1_0/1 -> butterfly2_0/1(a)
  node1_1/1 -> butterfly2_0/2(b)
  butterfly2_0/1(a+bw) -> node2_0/1
  butterfly2_0/2(a-bw) -> node2_1/1
  butterfly1_0/4(sync_out) -> butterfly2_0/3(sync)
  butterfly2_0/4(sync_out) -> sync_out/1
  slice1/1 -> butterfly2_0/4(shift), butterfly2_1/4(shift)
  butterfly2_0/3(of) -> of_2/1
  node1_2/1 -> butterfly2_1/1(a)
  node1_3/1 -> butterfly2_1/2(b)
  butterfly2_1/1(a+bw) -> node2_2/1
  butterfly2_1/2(a-bw) -> node2_3/1
  butterfly1_1/4(sync_out) -> butterfly2_1/3(sync)
  butterfly2_1/3(of) -> of_2/2

== system fft_wideband_real_test/fft_wideband_real/fft_unscrambler ==
  sync : Inport  OutDataType=sfix(16)  OutScaling=2^0
  In1 : Inport  Port=2  OutDataType=sfix(16)  OutScaling=2^0
  In2 : Inport  Port=3  OutDataType=sfix(16)  OutScaling=2^0
  const : xbsIndex_r4/Constant  arith_type=Boolean  const=1  n_bits=1  bin_pt=0  explicit_period=on  period=1  equ=P=C  opselect=C  inp2=PCIN>>17  opr=+  inp1=P  carry=CIN  dbl_ovrd=off  block_type=constant
      settings: block_version=9.1.01
  reorder : Subsystem  AncestorBlock=casper_library_reorder/reorder  mask(reorder){map=getfield( getfield( get_param( gcb,'UserData' ), 'parameters'),'map'), n_inputs=2, bram_latency=1, map_latency=1, double_buffer=0}
      mask prompts: map "Output Order:"; n_inputs "Number of inputs"; bram_latency "BRAM Latency"; map_latency "Map Latency"; double_buffer "Double Buffer"
      mask init:
      | reorder_init(gcb, ...
      |     'map', map, ...
      |     'n_inputs', n_inputs, ...
      |     'bram_latency', bram_latency, ...
      |     'map_latency', map_latency, ...
      |     'double_buffer', double_buffer);
      settings: AttributesFormatString=order=3
  square_transposer : Subsystem  AncestorBlock=casper_library_reorder/square_transposer  mask(square_transposer){n_inputs=1}
      mask prompts: n_inputs "Number of inputs (2^?):"
      mask init:
      | square_transposer_init(gcb,...
      |     'n_inputs', n_inputs);
      settings: AttributesFormatString=n_inputs=1
  sync_out : Outport  OutDataType=sfix(16)  OutScaling=2^0
  Out1 : Outport  Port=2  OutDataType=sfix(16)  OutScaling=2^0
  Out2 : Outport  Port=3  OutDataType=sfix(16)  OutScaling=2^0
  wires:
  sync/1 -> square_transposer/1(sync)
  square_transposer/1(sync_out) -> reorder/1(sync)
  reorder/1(sync_out) -> sync_out/1
  const/1 -> reorder/2(en)
  In1/1 -> square_transposer/2(In1)
  square_transposer/2(Out1) -> reorder/3(din0)
  reorder/3(dout0) -> Out1/1
  In2/1 -> square_transposer/3(In2)
  square_transposer/3(Out2) -> reorder/4(din1)
  reorder/4(dout1) -> Out2/1
